simulink model "SpeedController"  (R2026b)
settings: Solver=VariableStepAuto
values from neighbouring files (symbols this model uses):
  Duty_Coulomb = 1.024    [DCMotorParams.m]
  Duty_Max = 100    [DCMotorParams.m]
  Duty_StictionBoost = 9.0    (= 9)    [DCMotorParams.m]
  FF_Enable = 1    [DCMotorParams.m]
  Ki_Speed = 0.3778    [DCMotorParams.m]    (also in SpeedPI_design.mat = 0.377793746421; design_SpeedPI.m = res.Ki(sel))
  Kp_Speed = 0.01617    [DCMotorParams.m]    (also in SpeedPI_design.mat = 0.0161678564134; design_SpeedPI.m = res.Kp(sel))
  Stick_RPM = 5    [DCMotorParams.m]
  Ts = 0.01    [DCMotorParams.m]
libraries: simulink x1, slpidlib x1
settings Model: Creator=bence  LastModifiedBy=bence

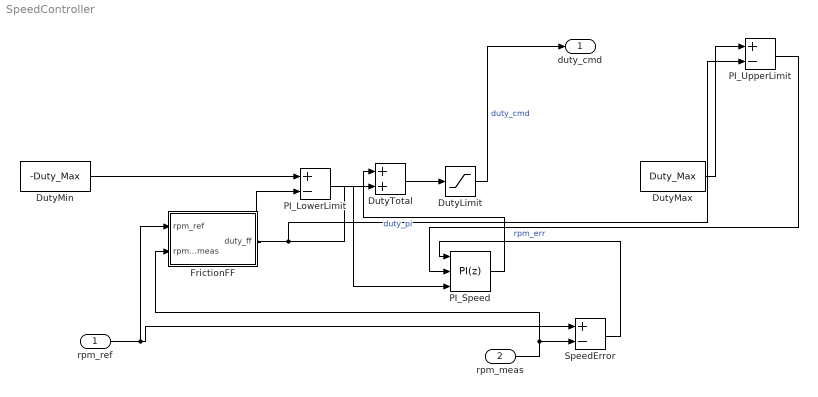
== system SpeedController ==
  rpm_ref : Inport
  rpm_meas : Inport  Port=2
  DutyLimit : Saturate  UpperLimit=Duty_Max  LowerLimit=-Duty_Max
  DutyMax : Constant  Value=Duty_Max
  DutyMin : Constant  Value=-Duty_Max
  DutyTotal : Sum
  FrictionFF : Subsystem
  PI_LowerLimit : Sum  Inputs=+-
  PI_Speed : slpidlib/PID Controller  Controller=PI  Form=Parallel  TimeDomain=Discrete-time  UseExternalTs=off  SampleTime=Ts  IntegratorMethod=Forward Euler  FilterMethod=Forward Euler  ControllerParametersSource=internal  P=Kp_Speed  I=Ki_Speed  UseKiTs=off  D=0  UseExternalDerivativeSource=off  N=100  UseFilter=on  TunerSelectOption=Transfer Function Based (PID Tuner App)  InitialConditionSource=internal  InitialConditionForIntegrator=0  InitialConditionForFilter=0  DifferentiatorICPrevScaledInput=0  ExternalReset=none  TrackingMode=off  Kt=1  LimitOutput=on  SatLimitsSource=external  UpperSaturationLimit=Duty_Max  LowerSaturationLimit=-Duty_Max  LinearizeAsGain=off  AntiWindupMode=clamping  Kb=1  LimitIntegrator=off  UpperIntegratorSaturationLimit=inf  LowerIntegratorSaturationLimit=-inf  POutMin=[]  POutMax=[]  IOutMin=[]  IOutMax=[]  DOutMin=[]  DOutMax=[]  NOutMin=[]  NOutMax=[]  SumOutMin=[]  SumOutMax=[]  SaturationOutMin=[]  SaturationOutMax=[]  PParamMin=[]  PParamMax=[]  IParamMin=[]  IParamMax=[]  DParamMin=[]  DParamMax=[]  NParamMin=[]  NParamMax=[]  KbParamMin=[]  KbParamMax=[]  KtParamMin=[]  KtParamMax=[]  KbOutMin=[]  KbOutMax=[]  KtOutMin=[]  KtOutMax=[]  IntegratorOutMin=[]  IntegratorOutMax=[]  FilterOutMin=[]  FilterOutMax=[]  SumI1OutMin=[]  SumI1OutMax=[]  SumI2OutMin=[]  SumI2OutMax=[]  SumI3OutMin=[]  SumI3OutMax=[]  SumI4OutMin=[]  SumI4OutMax=[]  SumDOutMin=[]  SumDOutMax=[]  DifferentiatorOutMin=[]  DifferentiatorOutMax=[]  FilterDiffOutCoefMin=[]  FilterDiffOutCoefMax=[]  ReciprocalOutMin=[]  ReciprocalOutMax=[]  SumDenOutMin=[]  SumDenOutMax=[]  SumNumOutMin=[]  SumNumOutMax=[]  DivideOutMin=[]  DivideOutMax=[]  UdiffTsProdOutMin=[]  UdiffTsProdOutMax=[]  NTsProdOutMin=[]  NTsProdOutMax=[]  UintegralTsProdOutMin=[]  UintegralTsProdOutMax=[]  UngainTsProdOutMin=[]  UngainTsProdOutMax=[]  ClampingZeroOutDataTypeStr=Inherit: Inherit via back propagation  ClampingZeroOutMin=[]  ClampingZeroOutMax=[]  FilterDenConstantOutDataTypeStr=Inherit: Inherit via back propagation  FilterDenConstantOutMin=[]  FilterDenConstantOutMax=[]  PCopyOutDataTypeStr=Inherit: Inherit via back propagation  PCopyOutMin=[]  PCopyOutMax=[]  NCopyOutDataTypeStr=Inherit: Inherit via back propagation  NCopyOutMin=[]  NCopyOutMax=[]  IntegratorContinuousStateAttributes=''  IntegratorStateMustResolveToSignalObject=off  IntegratorRTWStateStorageClass=Auto  FilterContinuousStateAttributes=''  FilterStateMustResolveToSignalObject=off  FilterRTWStateStorageClass=Auto  ParallelPVariant=InternalParameters  IdealPVariant=Disabled  IVariant=InternalParameters  DVariant=Disabled  IntegratorVariant=Discrete  SatVariant=External  AWVariant=DiscClampingParallel  PCopyVariant=Disabled  TRVariant=Disabled  FdbkBlocksVariant=Forward  IdealPFdbkVariant=Disabled  SatFdbkVariant=Disabled  DerivativeFilterVariant=Disabled  NVariant=Disabled  NCopyVariant=Disabled_SignalSpec  FilterICVariant=Disabled  IntegratorICVariant=InternalICs  ExternalResetVariant=Disabled  TRSumVariant=Passthrough  SumFdbkVariant=Disabled  SumVariant=Sum_PI  TsampFilterVariant=InternalTs  TsampNgainVariant=Passthrough  TsampIntegralVariant=Disabled_SignalSpec  ExternalSaturationOutDataTypeStr=Inherit: Same as second input  DerivativeSourceVariant=Disabled  PreIntVariant=InternalPreInt
      settings: LibrarySourceBlock=hdlsllib/Discrete/Discrete PID Controller
  PI_UpperLimit : Sum  Inputs=+-
  SpeedError : Sum  Inputs=+-
  duty_cmd : Outport
  wires:
  DutyMax/1 -> PI_UpperLimit/1
  DutyLimit/1 -> duty_cmd/1  "duty_cmd"
  DutyMin/1 -> PI_LowerLimit/1
  FrictionFF/1(duty_ff) -> PI_LowerLimit/2, PI_UpperLimit/2, DutyTotal/2
  rpm_ref/1 -> SpeedError/1, FrictionFF/1(rpm_ref)
  DutyTotal/1 -> DutyLimit/1
  PI_LowerLimit/1 -> PI_Speed/3
  rpm_meas/1 -> FrictionFF/2(rpm_meas), SpeedError/2
  PI_UpperLimit/1 -> PI_Speed/2
  SpeedError/1 -> PI_Speed/1  "rpm_err"
  PI_Speed/1 -> DutyTotal/1  "duty_pi"

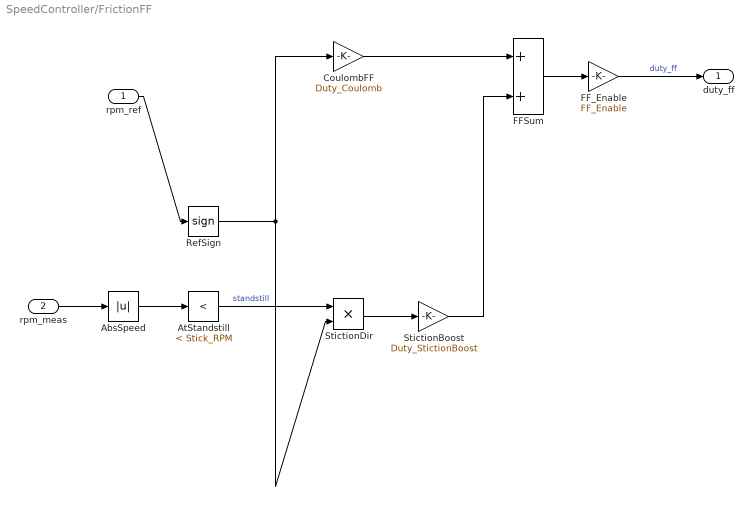
== system SpeedController/FrictionFF ==
  rpm_ref : Inport
  rpm_meas : Inport  Port=2
  AbsSpeed : Abs  SaturateOnIntegerOverflow=off
  AtStandstill : simulink/Logic and Bit Operations/Compare To Constant  relop=<  const=Stick_RPM  OutDataTypeStr=boolean
  CoulombFF : Gain  Gain=Duty_Coulomb
  FFSum : Sum
  FF_Enable : Gain  Gain=FF_Enable
  RefSign : Signum
  StictionBoost : Gain  Gain=Duty_StictionBoost
  StictionDir : Product
  duty_ff : Outport
  wires:
  RefSign/1 -> CoulombFF/1, StictionDir/2
  rpm_ref/1 -> RefSign/1
  CoulombFF/1 -> FFSum/1
  StictionDir/1 -> StictionBoost/1
  AtStandstill/1 -> StictionDir/1  "standstill"
  AbsSpeed/1 -> AtStandstill/1
  rpm_meas/1 -> AbsSpeed/1
  StictionBoost/1 -> FFSum/2
  FFSum/1 -> FF_Enable/1
  FF_Enable/1 -> duty_ff/1  "duty_ff"
